simulink model "planta"  (R2025b)
settings: Solver=ode3  StartTime=0.0  StopTime=inf  FixedStep=0.001  RelTol=1e-3
values from neighbouring files (symbols this model uses):
  ah_max = 0.75    [init_plant_parameters.m]
  at_max = 0.80    (= 0.8)    [init_plant_parameters.m]
  bcx = 1.0e6    (= 1000000)    [init_plant_parameters.m]
  bcy = 10.0e6    (= 10000000)    [init_plant_parameters.m]
  bh_eq = bhm+bhd/ih^2    (= 18.0165289256)    [init_plant_parameters.m]
  bhb = 100e6    (= 100000000)    [init_plant_parameters.m]
  bhEb = 2.2e9    (= 2200000000)    [init_plant_parameters.m]
  bhwu = 150    [init_plant_parameters.m]
  bt = 90.0    (= 90)    [init_plant_parameters.m]
  bt_eq = btm+btd/it^2    (= 6.002)    [init_plant_parameters.m]
  btb = 5.0e6    (= 5000000)    [init_plant_parameters.m]
  btw = 3.0e3    (= 3000)    [init_plant_parameters.m]
  counter_limit = timeout/(Ts0*1000)    (= 1500)    [init_plant_parameters.m]
  envolvent = [ones(1,N_xt)]*38    [init_plant_parameters.m]
  g = 9.80665    [init_plant_parameters.m]
  Hc = 2.59    [init_plant_parameters.m]
  ih = 22.0    (= 22)    [init_plant_parameters.m]
  it = 30.0    (= 30)    [init_plant_parameters.m]
  Jh_eq = Jhm_hb+Jhd_hEb/ih^2    (= 37.8512396694)    [init_plant_parameters.m]
  Jt_eq = Jtm_tb+Jtd/it^2    (= 8.33333333333)    [init_plant_parameters.m]
  k_i_c = abs(polos_obs_c)^3    [init_plant_parameters.m]
  k_i_h = abs(polos_obs_h)^3    [init_plant_parameters.m]
  k_omega_c = 3 * abs(polos_obs_c)^2    [init_plant_parameters.m]
  k_omega_h = 3 * abs(polos_obs_h)^2-k_tita_h*bh_eq/Jh_eq    [init_plant_parameters.m]
  k_tita_c = 3 * abs(polos_obs_c)    [init_plant_parameters.m]
  k_tita_h = 3 * abs(polos_obs_h)-bh_eq/Jh_eq    [init_plant_parameters.m]
  Kcy = 1.8e9    (= 1800000000)    [init_plant_parameters.m]
  khwu = 236e6    (= 236000000)    [init_plant_parameters.m]
  Ki_c = (wn_t^2*Mt)/Kf    (= 320)    [init_plant_parameters.m]
  Ki_i = (wn_h^2)*Jh_eq    (= 2422.47933884)    [init_plant_parameters.m]
  Kp_c = (2*zitta_t*wn_t*Mt)/Kf    (= 1120)    [init_plant_parameters.m]
  Kp_i = 2*zitta_h*wn_h*Jh_eq    (= 1211.23966942)    [init_plant_parameters.m]
  Ktw = 480e3    (= 480000)    [init_plant_parameters.m]
  Lh0 = 110    [init_plant_parameters.m]
  lh_0 = Yt0-yh_0    (= 7)    [init_plant_parameters.m]
  Mc_max = 50000    [init_plant_parameters.m]
  Mc_min = 2000    [init_plant_parameters.m]
  Ms = 15000    [init_plant_parameters.m]
  Mt = 30000    [init_plant_parameters.m]
  P_nom = 956150    [init_plant_parameters.m]
  periodo_pulsos = 100    [init_plant_parameters.m]
  rhd = 0.75    [init_plant_parameters.m]
  rtd = 0.50    (= 0.5)    [init_plant_parameters.m]
  tau_hm = Ts2    (= 0.001)    [init_plant_parameters.m]
  tau_tm = Ts2    (= 0.001)    [init_plant_parameters.m]
  Thb_Max = 50e3    (= 50000)    [init_plant_parameters.m]
  ThEb_Max = 1.1e6    (= 1100000)    [init_plant_parameters.m]
  Thm_0 = 0    [init_plant_parameters.m]
  Thm_Max = 20e3    (= 20000)    [init_plant_parameters.m]
  titahm_0 = yl_0/(rhd/(2*ih))    (= 2228.19975108)    [init_plant_parameters.m]
  titatm_0 = xtd_0/(rtd/it)    (= 300)    [init_plant_parameters.m]
  Ts0 = 0.02    [init_plant_parameters.m]
  Ts1 = 0.02    [init_plant_parameters.m]
  Ttb_Max = 5.0e3    (= 5000)    [init_plant_parameters.m]
  Ttm_0 = 0    [init_plant_parameters.m]
  Ttm_Max = 4.0e3    (= 4000)    [init_plant_parameters.m]
  vh_0 = 0    [init_plant_parameters.m]
  vh_max = 3    [init_plant_parameters.m]
  vh_nom = 1.5    [init_plant_parameters.m]
  vt_0 = 0    [init_plant_parameters.m]
  vt_max = 4.0    (= 4)    [init_plant_parameters.m]
  Wc = 2.44    [init_plant_parameters.m]
  x_LIDAR = 3    [init_plant_parameters.m]
  xl_0 = 5    [init_plant_parameters.m]
  xt_0 = 5    [init_plant_parameters.m]
  xt_max = 50.0    (= 50)    [init_plant_parameters.m]
  xt_min = -30.0    (= -30)    [init_plant_parameters.m]
  xtd_0 = xt_0    (= 5)    [init_plant_parameters.m]
  yc0_vec_inicial = [ 0, 0, 1, 0, 0, 1, 0, 0, 0, 0, 0, 0, alt_borde,                   3, 5, 6, 3, 5, 6, 6, 4, 1, 1, -4, -5, -2, -1, 2, 6, 4, 2, 5,                   alt_borde] * Hc    [init_plant_parameters.m]
  yh_max = 40    [init_plant_parameters.m]
  yh_min = -20    [init_plant_parameters.m]
  yl_0 = Yt0 - l_0    (= 37.9806775752)    [init_plant_parameters.m]
  Yt0 = 45.0    (= 45)    [init_plant_parameters.m]
  zitta = 0.5    [init_plant_parameters.m]
undefined symbols (not defined in the file or in its folder): DiscIntNeverNeededParam
libraries: sl3dlib x1, dspnetwork x1
(part 1 of 2)
settings Model: SimulationMode=accelerator  PacingRate=2  Creator=lauta  LastModifiedBy=bruno

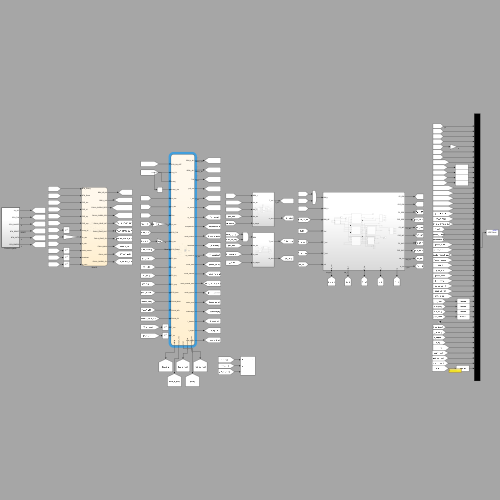
[thumbnail: Simulink's stored preview of the top-level diagram]
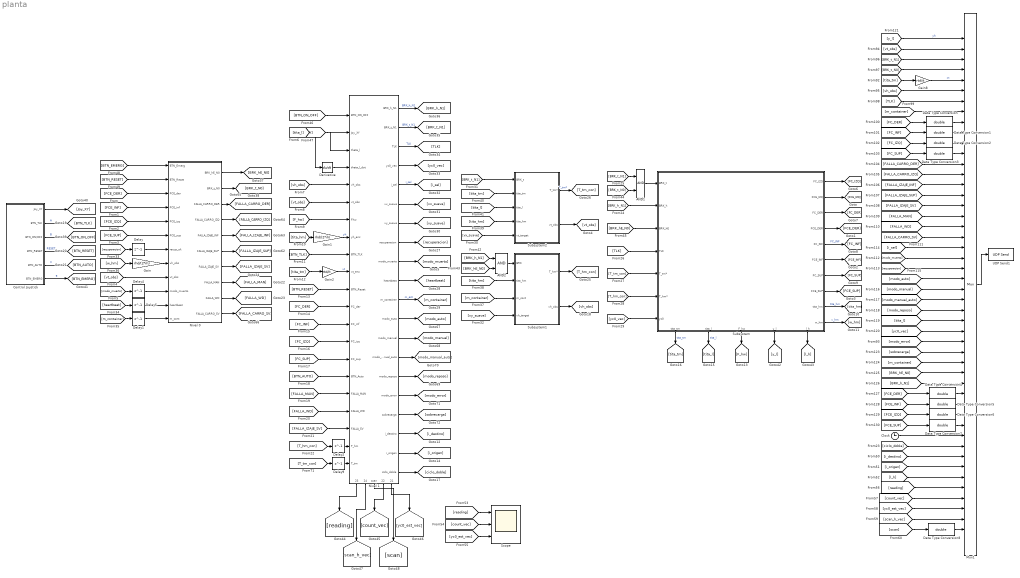
== system planta ==
  AND1 : Logic  IconShape=distinctive  AllPortsSameDT=off  OutDataTypeStr=boolean
  AND2 : Logic  IconShape=distinctive  AllPortsSameDT=off  OutDataTypeStr=boolean
  Clock : Clock
  "Control Joystick " : Subsystem  TreatAsAtomicUnit=on  SystemSampleTime=tau_hm
  Data Type Conversion{,1..8} (9 alike) : DataTypeConversion  OutDataTypeStr=double  SaturateOnIntegerOverflow=off  RndMeth=Floor
  Delay{,1..2,4..5,9} (6 alike) : Delay  DelayLength=1  InputProcessing=Columns as channels (frame based)  SampleTime=Ts0
  Derivative : Derivative
  Gain : Gain  Gain=rhd/(2*ih)
  Gain1 : Gain  Gain=rhd/(2*ih)
  Gain2 : Gain  Gain=rtd/it
  Gain8 : Gain  Gain=rtd/it
  Mux1 : Mux  Inputs=48
  Nivel 0 : Stateflow chart  TreatAsAtomicUnit=on  SystemSampleTime=Ts0
  Nivel 1 : Stateflow chart  TreatAsAtomicUnit=on  SystemSampleTime=Ts1
      settings: PortSchema="{\"entries\":[{\"content\":{\"sides\":[{\"content\":{\"connectorIds\":[\"In1\",\"In2\",\"In3\",\"In4\",\"In5\",\"In6\",\"In7\",\"In8\",\"In9\",\"In10\",\"In11\",\"In12\",\"In13\",\"In14\",\"In15\",\"In16\",\"In17\",\"In18\",\"In19\",\"In20\",\"In21\"]},\"type\":\"ConnectorPlacement.EquallySpacedRectSide\",\"uuid\":\"f9309f7f-3c54-46e4-8c5b-2437500e737a\"},{\"content\":{\"connectorIds\":[\"Out1\",\"Out2\",\"Out3\",\"Out4\",\"Out5\",\"Out6\",\"Out7\",\"Out8\",\"Out9\",\"Out10\",\"Out11\",\"Out12\",\"Out13\",\"Out14\",\"Out15\",\"Out16\",\"Out17\",\"Out18\",\"Out19\",\"Out20\"],\"side\":\"RIGHT\"},\"type\":\"ConnectorPlacement.EquallySpacedRectSide\",\"uuid\":\"ccb321bc-00c9-4449-9a3e-5435c9b39512\"},{\"content\":{\"side\":\"TOP\"},\"type\":\"ConnectorPlacement.EquallySpacedRectSide\",\"uuid\":\"3099bf00-db3f-4e40-be81-3cc0981b79ca\"},{\"content\":{\"connectorIds\":[\"Out23\",\"Out24\",\"Out25\",\"Out22\",\"Out21\"],\"side\":\"BOTTOM\"},\"type\":\"ConnectorPlacement.EquallySpacedRectSide\",\"uuid\":\"36423b9f-354b-4379-ba2c-4a5a21c34b61\"}]},\"type\":\"ConnectorPlacement.EquallySpacedConnector\",\"uuid\":\"738d8a71-e82f-4c2f-ab09-6d96e2c2ffc9\"}],\"packageUris\":[\"http://schema.mathworks.com/mf0/Connector/R2020b\"],\"version\":\"1.0\"}"
  Scope : Scope  NumInputPorts=3
      settings: ActiveDisplayYMinimum=-212.88770278621519  ActiveDisplayYMaximum=339.27135541787879
  Subsystem : Subsystem
      settings: PortSchema="{\"entries\":[{\"content\":{\"sides\":[{\"content\":{\"connectorIds\":[\"In1\",\"In2\",\"In3\",\"In4\",\"In5\",\"In6\",\"In7\"]},\"type\":\"ConnectorPlacement.EquallySpacedRectSide\",\"uuid\":\"af149f61-d672-449c-a7fb-5624cb810af3\"},{\"content\":{\"connectorIds\":[\"Out1\",\"Out2\",\"Out3\",\"Out4\",\"Out5\",\"Out6\",\"Out7\",\"Out8\",\"Out9\",\"Out10\"],\"side\":\"RIGHT\"},\"type\":\"ConnectorPlacement.EquallySpacedRectSide\",\"uuid\":\"108c8060-9c99-461a-9367-2154718b4d28\"},{\"content\":{\"side\":\"TOP\"},\"type\":\"ConnectorPlacement.EquallySpacedRectSide\",\"uuid\":\"cb8fd5b9-c875-48a1-bd6c-0e8918880b0e\"},{\"content\":{\"connectorIds\":[\"Out11\",\"Out12\",\"Out13\",\"Out14\",\"Out15\"],\"side\":\"BOTTOM\"},\"type\":\"ConnectorPlacement.EquallySpacedRectSide\",\"uuid\":\"417db1a2-cc41-4820-881b-53f0e9bd83f8\"}]},\"type\":\"ConnectorPlacement.EquallySpacedConnector\",\"uuid\":\"d40848f9-2d56-455f-ab83-092311f7e026\"}],\"packageUris\":[\"http://schema.mathworks.com/mf0/Connector/R2020b\"],\"version\":\"1.0\"}"
  Subsystem1 : Subsystem
  Subsystem2 : Subsystem
  UDP Send1 : dspnetwork/UDP Send  remoteURL='127.0.0.1'  remotePort=1234  localURL='0.0.0.0'  localPortSource=Automatically determine  localPort=-1  sendBufferSize=8192  sampletime=-1  blockPlatform=HOST  separateLengthPort=0
  wires:
  Subsystem2/1(T_tm*) -> [T_tm_con]  "T_tm*"
  Subsystem/12(tita_l) -> [tita_l]  "tita_l"
  Subsystem1/1(T_hm*) -> [T_hm_con]
  Subsystem/11(tita_tm) -> [tita_tm]  "tita_tm"
  Subsystem/9(tita_hm) -> [tita_hm]  "tita_hm"
  Nivel 1/1(BRK_h_N1) -> [BRK_h_N1]  "BRK_h_N1"
  Nivel 1/2(BRK_t_N1) -> [BRK_t_N1]  "BRK_t_N1"
  "Control Joystick "/1(Joy_XY) -> [Joy_XY]
  Subsystem2/2(vt_obs) -> [vt_obs]
  Subsystem1/2(vh_obs) -> [vh_obs]
  Derivative/1 -> Nivel 1/4(theta_l_dot)
  Subsystem/13(F_hw) -> [F_hw]
  Nivel 1/3(TLK) -> [TLK]  "TLK"
  "Control Joystick "/2(BTN_TLK) -> [BTN_TLK]  "A"
  Nivel 1/4(yc0_vec) -> [yc0_vec]
  Nivel 1/11(m_container) -> [m_container]  "m_est"
  "Control Joystick "/4(BTN_RESET) -> [BTN_RESET]  "RESET"
  Subsystem/3(FC_DER) -> [FC_DER]
  Subsystem/5(FC_INF) -> [FC_INF]  "FC_INF"
  Subsystem/7(FC_SUP) -> [FC_SUP]
  "Control Joystick "/5(BTN_AUTO) -> [BTN_AUTO]  "X"
  Nivel 1/6(vx_suave) -> [vx_suave]
  Nivel 1/7(vy_suave) -> [vy_suave]
  "Control Joystick "/6(BTN_EMERG) -> [BTN_EMERG]  "9"
  Nivel 1/8(recuperacion) -> [recuperacion]
  Subsystem/10(w_hm) -> [w_hm]  "v_hm"
  Gain/1 -> Nivel 0/8(vh_obs)
  AND1/1 -> Subsystem/1(BRK_t)
  Nivel 0/2(BRK_t_N0) -> [BRK_t_N0]
  Subsystem/2(FCE_IZQ) -> [FCE_IZQ]
  Subsystem/4(FCE_DER) -> [FCE_DER]
  Subsystem/6(FCE_INF) -> [FCE_INF]
  Subsystem/8(FCE_SUP) -> [FCE_SUP]
  [FCE_DER] -> Nivel 0/3(FCE_der)
  [FCE_INF] -> Nivel 0/4(FCE_inf)
  [FCE_IZQ] -> Nivel 0/5(FCE_izq)
  [FCE_SUP] -> Nivel 0/6(FCE_sup)
  Nivel 0/8(FALLA_MAN) -> [FALLA_MAN]
  Nivel 0/9(FALLA_WD) -> [FALLA_WD]
  Nivel 0/7(FALLA_IZAJE_SV) -> [FALLA_IZAJE_SV]
  Delay/1 -> Nivel 0/7(recup_ok)
  Delay1/1 -> Nivel 0/12(m_cont)
  [vt_obs] -> Nivel 0/9(vt_obs)
  "Control Joystick "/3(BTN_ON/OFF) -> [BTN_ON_OFF]  "B"
  Delay2/1 -> Nivel 1/20(T_hm)
  Delay9/1 -> Nivel 1/21(T_tm)
  Nivel 1/9(modo_muerto) -> [modo_muerto]
  [modo_muerto] -> Delay4/1
  Nivel 1/10(heartbeat) -> [heartbeat]
  Delay4/1 -> Nivel 0/10(modo_muerto)
  Delay5/1 -> Nivel 0/11(heartbeat)
  [tita_l] -> Derivative/1, Nivel 1/3(theta_l)
  [vh_obs] -> Nivel 1/5(vh_obs)
  [vt_obs] -> Nivel 1/6(vt_obs)
  [F_hw] -> Nivel 1/7(Fhw)
  [tita_hm] -> Gain1/1
  Gain1/1 -> Nivel 1/8(yh_enc)  "yh"
  [BTN_TLK] -> Nivel 1/9(BTN_TLK)
  [tita_tm] -> Gain2/1
  Gain2/1 -> Nivel 1/10(xt_enc)  "xt"
  [BTN_RESET] -> Nivel 1/11(BTN_Reset)
  [FC_DER] -> Nivel 1/12(FC_der)
  [FC_INF] -> Nivel 1/13(FC_inf)
  [FC_IZQ] -> Nivel 1/14(FC_izq)
  [FC_SUP] -> Nivel 1/15(FC_sup)
  [BTN_AUTO] -> Nivel 1/16(BTN_Auto)
  [FALLA_MAN] -> Nivel 1/17(FALLA_MAN)
  [FALLA_WD] -> Nivel 1/18(FALLA_WD)
  [FALLA_IZAJE_SV] -> Nivel 1/19(FALLA_SV)
  [T_hm_con] -> Delay2/1
  [T_tm_con] -> Delay9/1
  Nivel 1/5(i_sel) -> [i_sel]  "i_sel"
  [BRK_h_N1] -> Subsystem/2(BRK_h)
  [BRK_t_N1] -> AND1/1
  [TLK] -> Subsystem/4(TLK)
  [T_tm_con] -> Subsystem/5(T_tm*)
  [T_hm_con] -> Subsystem/6(T_hm*)
  [yc0_vec] -> Subsystem/7(yc0)
  [vx_suave] -> Subsystem2/5(vt_target)
  [BRK_t_N1] -> Subsystem2/1(BRK_t)
  [vy_suave] -> Subsystem1/4(vh_target)
  [recuperacion] -> Delay/1
  [heartbeat] -> Delay5/1
  [m_container] -> Delay1/1
  [w_hm] -> Gain/1
  [m_container] -> Subsystem1/3(m_cont)
  [tita_hm] -> Subsystem1/2(tita_hm)
  [tita_hm] -> Subsystem2/4(tita_hm)
  [tita_tm] -> Subsystem2/2(tita_tm)
  [tita_l] -> Subsystem2/3(tita_l)
  [BRK_h_N1] -> AND2/1
  AND2/1 -> Subsystem1/1(BRK)
  Nivel 0/1(BRK_hE_N0) -> [BRK_hE_N0]
  [BRK_hE_N0] -> AND2/2
  [BRK_t_N0] -> AND1/2
  [BRK_hE_N0] -> Subsystem/3(BRK_hE)
  [BTN_ON_OFF] -> Nivel 1/1(BTN_ON_OFF)
  [Joy_XY] -> Nivel 1/2(Joy_XY)
  [BTN_EMERG] -> Nivel 0/1(BTN_Emerg)
  [BTN_RESET] -> Nivel 0/2(BTN_Reset)
  Subsystem/14(y_l) -> [y_l]
  Nivel 0/3(FALLA_CARRO_DER) -> [FALLA_CARRO_DER]
  Nivel 0/4(FALLA_CARRO_IZQ) -> [FALLA_CARRO_IZQ]
  Nivel 0/5(FALLA_IZAJE_INF) -> [FALLA_IZAJE_INF]
  Nivel 0/6(FALLA_IZAJE_SUP) -> [FALLA_IZAJE_SUP]
  Nivel 0/10(FALLA_CARRO_SV) -> [FALLA_CARRO_SV]
  Mux1/1 -> UDP Send1/1
  Nivel 1/12(modo_auto) -> [modo_auto]
  Nivel 1/13(modo_manual) -> [modo_manual]
  Nivel 1/14(modo_manual_auto) -> [modo_manual_auto]
  Nivel 1/15(modo_reposo) -> [modo_reposo]
  [y_l] -> Mux1/1  "yh"
  [vt_obs] -> Mux1/2
  [BRK_t_N1] -> Mux1/3
  [BRK_t_N0] -> Mux1/4
  [vh_obs] -> Mux1/6
  [TLK] -> Mux1/7
  [m_container] -> Mux1/8
  [FC_INF] -> Data Type Conversion1/1
  [FC_SUP] -> Data Type Conversion3/1
  [FALLA_CARRO_DER] -> Mux1/13
  [FALLA_CARRO_IZQ] -> Mux1/14
  [FALLA_IZAJE_INF] -> Mux1/15
  [FALLA_IZAJE_SUP] -> Mux1/16
  [FALLA_IZAJE_SV] -> Mux1/17
  [FALLA_MAN] -> Mux1/18
  [FALLA_WD] -> Mux1/19
  [FALLA_CARRO_SV] -> Mux1/20
  [i_sel] -> Mux1/21
  [modo_muerto] -> Mux1/22
  [recuperacion] -> Mux1/23
  [modo_auto] -> Mux1/24
  [modo_manual] -> Mux1/25
  [modo_manual_auto] -> Mux1/26
  [modo_reposo] -> Mux1/27
  [tita_tm] -> Gain8/1
  Gain8/1 -> Mux1/5  "xt"
  [FC_IZQ] -> Data Type Conversion2/1
  [FC_DER] -> Data Type Conversion/1
  Data Type Conversion/1 -> Mux1/9
  Subsystem/1(FC_IZQ) -> [FC_IZQ]
  Data Type Conversion1/1 -> Mux1/10
  Data Type Conversion2/1 -> Mux1/11
  Data Type Conversion3/1 -> Mux1/12
  [tita_l] -> Mux1/28
  [yc0_vec] -> Mux1/29
  Nivel 1/16(modo_error) -> [modo_error]
  [modo_error] -> Mux1/30
  Nivel 1/17(sobrecarga) -> [sobrecarga]
  [sobrecarga] -> Mux1/31
  [m_container] -> Mux1/32
  [BRK_hE_N0] -> Mux1/33
  [BRK_h_N1] -> Mux1/34
  [FCE_DER] -> Data Type Conversion4/1
  [FCE_INF] -> Data Type Conversion5/1
  [FCE_IZQ] -> Data Type Conversion6/1
  [FCE_SUP] -> Data Type Conversion7/1
  Data Type Conversion5/1 -> Mux1/36
  Data Type Conversion6/1 -> Mux1/37
  Data Type Conversion7/1 -> Mux1/38
  Data Type Conversion4/1 -> Mux1/35
  Clock/1 -> Mux1/39
  Nivel 1/18(i_destino) -> [i_destino]
  Nivel 1/19(i_origen) -> [i_origen]
  Nivel 1/20(ciclo_doble) -> [ciclo_doble]
  [ciclo_doble] -> Mux1/40
  [i_destino] -> Mux1/41
  [i_origen] -> Mux1/42
  Subsystem/15(l_h) -> [l_h]
  [l_h] -> Mux1/43
  [reading] -> Scope/1
  [count_vec] -> Scope/2
  [yc0_est_vec] -> Scope/3
  [reading] -> Mux1/44
  [count_vec] -> Mux1/45
  [yc0_est_vec] -> Mux1/46
  Nivel 1/23(reading) -> [reading]
  Nivel 1/22(count_vec) -> [count_vec]
  Nivel 1/21(yc0_est_vec) -> [yc0_est_vec]
  Nivel 1/24(scan_h_vec) -> [scan_h_vec]
  [scan_h_vec] -> Mux1/47
  Nivel 1/25(scan) -> [scan]
  [scan] -> Data Type Conversion8/1
  Data Type Conversion8/1 -> Mux1/48

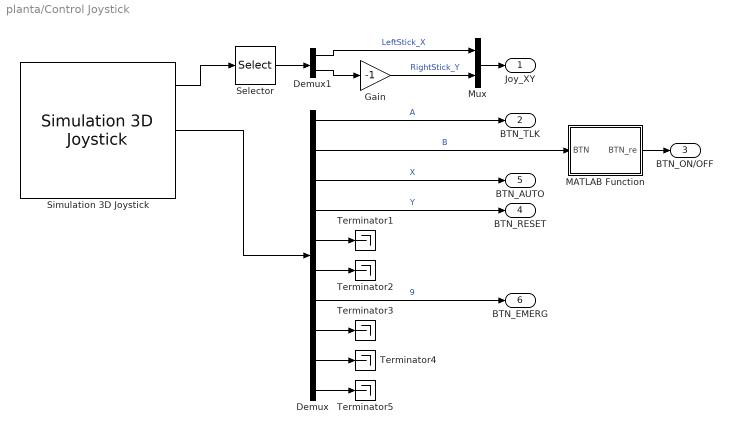
== system planta/Control Joystick  ==
  Demux : Demux  Outputs=10
  Demux1 : Demux  Outputs=2
  Gain : Gain  Gain=-1
  MATLAB Function : MATLAB Function  TreatAsAtomicUnit=on
  Mux : Mux  Inputs=2
  Selector : Selector  InputPortWidth=5  IndexOptions=Index vector (dialog)  Indices=[1 5]  OutputSizes=1
  Simulation 3D Joystick : sl3dlib/Simulation 3D/Hardware Interface/Simulation 3D Joystick  joyid=1  adjustports=on  forcefeed=off
  Terminator{1..5} (5 alike) : Terminator
  Joy_XY : Outport
  BTN_TLK : Outport  Port=2
  BTN_ON/OFF : Outport  Port=3
  BTN_RESET : Outport  Port=4
  BTN_AUTO : Outport  Port=5
  BTN_EMERG : Outport  Port=6
  wires:
  Demux/1 -> BTN_TLK/1  "A"
  Demux1/2 -> Gain/1
  Demux1/1 -> Mux/1  "LeftStick_X"
  Selector/1 -> Demux1/1
  Simulation 3D Joystick/1 -> Selector/1
  Gain/1 -> Mux/2  "RightStick_Y"
  Simulation 3D Joystick/2 -> Demux/1
  Demux/2 -> MATLAB Function/1(BTN)  "B"
  Demux/3 -> BTN_AUTO/1  "X"
  Demux/4 -> BTN_RESET/1  "Y"
  Mux/1 -> Joy_XY/1
  Demux/5 -> Terminator1/1
  Demux/6 -> Terminator2/1
  Demux/8 -> Terminator3/1
  Demux/9 -> Terminator4/1
  Demux/10 -> Terminator5/1
  Demux/7 -> BTN_EMERG/1  "9"
  MATLAB Function/1(BTN_re) -> BTN_ON/OFF/1

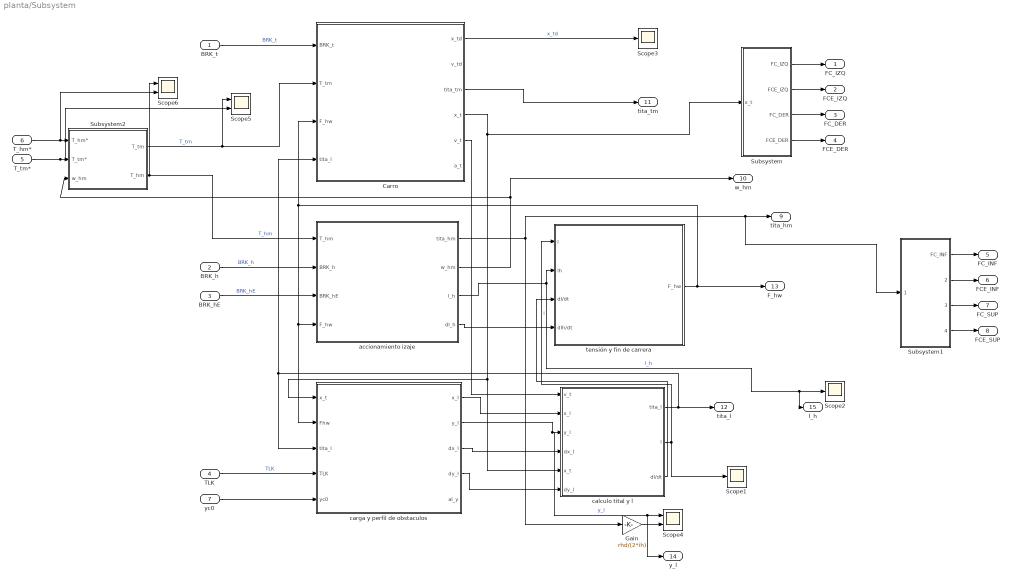
== system planta/Subsystem ==
  BRK_t : Inport
  BRK_h : Inport  Port=2
  BRK_hE : Inport  Port=3
  TLK : Inport  Port=4
  T_tm* : Inport  Port=5
  T_hm* : Inport  Port=6
  yc0 : Inport  Port=7
  Carro : Subsystem
  Gain : Gain  Gain=rhd/(2*ih)
  Scope1 : Scope
      settings: ActiveDisplayYMinimum=-3.1438  ActiveDisplayYMaximum=28.29416  DataLoggingVariableName=ScopeData5
  Scope2 : Scope
      settings: ActiveDisplayYMinimum=19.873309767116591  ActiveDisplayYMaximum=50.479762765379171  DataLoggingVariableName=ScopeData6
  Scope3 : Scope
      settings: ActiveDisplayYMinimum=-36.0687664182162  ActiveDisplayYMaximum=31.78541849091291
  Scope4 : Scope  NumInputPorts=2
      settings: ActiveDisplayYMinimum=31.554051944720545  ActiveDisplayYMaximum=41.717948866314323  DataLoggingVariableName=ScopeData13
  Scope5 : Scope  NumInputPorts=2
      settings: ActiveDisplayYMinimum=2216.0147211124222  ActiveDisplayYMaximum=3994.0783191721102  DataLoggingVariableName=ScopeData12
  Scope6 : Scope  NumInputPorts=2
      settings: ActiveDisplayYMinimum=-18675.827607289168  ActiveDisplayYMaximum=162181.63787626589  DataLoggingVariableName=ScopeData17
  Subsystem : Subsystem
  Subsystem1 : Subsystem
  Subsystem2 : Subsystem
  accionamiento izaje : Subsystem
  calculo tital y l : Subsystem
  carga y perfil de obstaculos : Subsystem
  tensión y fin de carrera : Subsystem
  FC_IZQ : Outport
  FCE_IZQ : Outport  Port=2
  FC_DER : Outport  Port=3
  FCE_DER : Outport  Port=4
  FC_INF : Outport  Port=5
  FCE_INF : Outport  Port=6
  FC_SUP : Outport  Port=7
  FCE_SUP : Outport  Port=8
  tita_hm : Outport  Port=9
  w_hm : Outport  Port=10
  tita_tm : Outport  Port=11
  tita_l : Outport  Port=12
  F_hw : Outport  Port=13
  y_l : Outport  Port=14
  l_h : Outport  Port=15
  wires:
  Subsystem2/2(T_hm) -> Scope6/1, accionamiento izaje/1(T_hm)  "T_hm"
  Carro/1(x_td) -> Scope3/1  "x_td"
  Carro/5(v_t) -> calculo tital y l/1(v_t)
  calculo tital y l/3(dl/dt) -> tensión y fin de carrera/3(dl/dt)
  carga y perfil de obstaculos/3(dx_l) -> calculo tital y l/4(dx_l)
  tensión y fin de carrera/1(F_hw) -> carga y perfil de obstaculos/2(Fhw), accionamiento izaje/4(F_hw), Carro/3(F_hw), F_hw/1
  carga y perfil de obstaculos/1(x_l) -> calculo tital y l/2(x_l)
  BRK_t/1 -> Carro/1(BRK_t)  "BRK_t"
  Subsystem2/1(T_tm) -> Scope5/1, Carro/2(T_tm)  "T_tm"
  BRK_hE/1 -> accionamiento izaje/3(BRK_hE)  "BRK_hE"
  BRK_h/1 -> accionamiento izaje/2(BRK_h)  "BRK_h"
  accionamiento izaje/3(l_h) -> l_h/1, Scope2/1, tensión y fin de carrera/2(lh)  "l_h"
  calculo tital y l/1(tita_l) -> tita_l/1, carga y perfil de obstaculos/3(tita_l), Carro/4(tita_l)
  carga y perfil de obstaculos/4(dy_l) -> calculo tital y l/6(dy_l)
  Carro/4(x_t) -> carga y perfil de obstaculos/1(x_t), calculo tital y l/5(x_t), Subsystem/1(x_t)
  carga y perfil de obstaculos/2(y_l) -> y_l/1, Scope4/1, calculo tital y l/3(y_l)  "y_l"
  calculo tital y l/2(l) -> Scope1/1, tensión y fin de carrera/1(l)  "l"
  accionamiento izaje/1(tita_hm) -> Gain/1, Subsystem1/1(tita_hm), tita_hm/1
  TLK/1 -> carga y perfil de obstaculos/4(TLK)  "TLK"
  Carro/3(tita_tm) -> tita_tm/1
  accionamiento izaje/2(w_hm) -> Subsystem2/3(w_hm), w_hm/1
  T_hm*/1 -> Scope6/2, Subsystem2/1(T_hm*)
  T_tm*/1 -> Scope5/2, Subsystem2/2(T_tm*)
  accionamiento izaje/4(dl_h) -> tensión y fin de carrera/4(dlh/dt)
  yc0/1 -> carga y perfil de obstaculos/5(yc0)
  Subsystem/1(FC_IZQ) -> FC_IZQ/1
  Subsystem/2(FCE_IZQ) -> FCE_IZQ/1
  Subsystem/3(FC_DER) -> FC_DER/1
  Subsystem/4(FCE_DER) -> FCE_DER/1
  Subsystem1/1(FC_INF) -> FC_INF/1
  Subsystem1/2(FCE_INF) -> FCE_INF/1
  Subsystem1/3(FC_SUP) -> FC_SUP/1
  Subsystem1/4(FCE_SUP) -> FCE_SUP/1
  Gain/1 -> Scope4/2

== system planta/Subsystem1 ==
  BRK : Inport
  tita_hm : Inport  Port=2
  m_cont : Inport  Port=3
  vh_target : Inport  Port=4
  Controlador de Velocidad : Subsystem  TreatAsAtomicUnit=on  SystemSampleTime=tau_hm
  Delay2 : Delay  DelayLength=1  InitialCondition=Thm_0
  Modulación de la Referencia : Subsystem  TreatAsAtomicUnit=on  SystemSampleTime=tau_tm
  Observador de estado : Subsystem  TreatAsAtomicUnit=on  SystemSampleTime=tau_hm
  Scope : Scope
      settings: ActiveDisplayYMinimum=-0.34044660881355743  ActiveDisplayYMaximum=0.29766878557385207  DataLoggingVariableName=ScopeData22
  Scope1 : Scope
      settings: ActiveDisplayYMinimum=2409.3798864876212  ActiveDisplayYMaximum=2546.7876456481149  DataLoggingVariableName=ScopeData23
  Scope2 : Scope
      settings: ActiveDisplayYMinimum=-0.0013706448423018264  ActiveDisplayYMaximum=0.0033174735734584049  DataLoggingVariableName=ScopeData24
  T_hm* : Outport
  vh_obs : Outport  Port=2
  wires:
  Delay2/1 -> Observador de estado/2(Thm_ref)
  Modulación de la Referencia/1(vh_ref) -> Scope/1, Controlador de Velocidad/3(vh_ref)
  m_cont/1 -> Controlador de Velocidad/1(m_container)
  BRK/1 -> Controlador de Velocidad/2(BRK)
  Controlador de Velocidad/1(T_hm*) -> Scope1/1, T_hm*/1, Delay2/1
  Observador de estado/1(vh_obs) -> Scope2/1, vh_obs/1, Controlador de Velocidad/4(vh_obs)
  tita_hm/1 -> Observador de estado/1(yh_enc)
  vh_target/1 -> Modulación de la Referencia/1(vh)

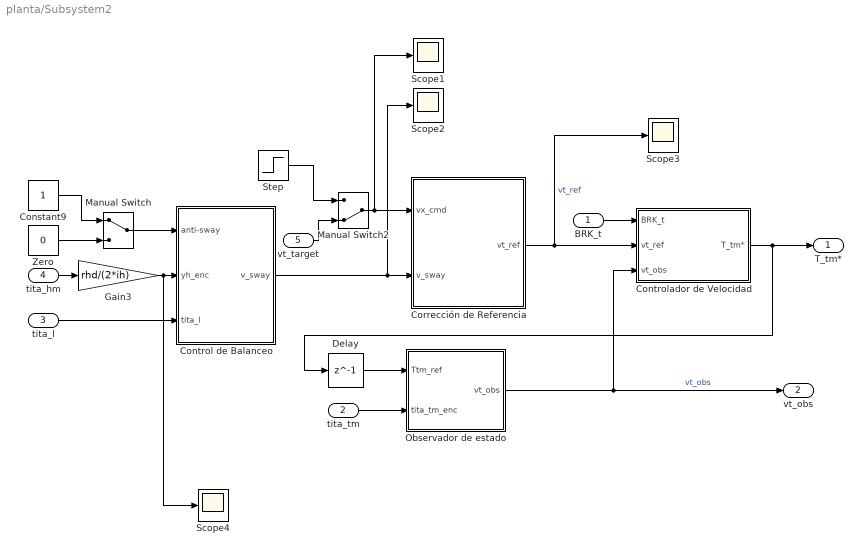
== system planta/Subsystem2 ==
  BRK_t : Inport
  tita_tm : Inport  Port=2
  tita_l : Inport  Port=3
  tita_hm : Inport  Port=4
  vt_target : Inport  Port=5
  Constant9 : Constant
  Control de Balanceo : Subsystem
  Controlador de Velocidad : Subsystem
  Corrección de Referencia : Subsystem
  Delay : Delay  DelayLength=1  InitialCondition=Ttm_0
  Gain3 : Gain  Gain=rhd/(2*ih)
  Manual Switch : ManualSwitch
  Manual Switch2 : ManualSwitch  CurrentSetting=0
  Observador de estado : Subsystem  TreatAsAtomicUnit=on  SystemSampleTime=tau_hm
  Scope{1..4} (4 alike) : Scope
      Scope1 settings: ActiveDisplayYMinimum=-0.5858905301065096  ActiveDisplayYMaximum=1.1762100589007232  DataLoggingVariableName=ScopeData14
      Scope2 settings: ActiveDisplayYMinimum=-0.71026747882004693  ActiveDisplayYMaximum=0.0886681616928574  DataLoggingVariableName=ScopeData15
      Scope3 settings: ActiveDisplayYMinimum=-0.6534407131284351  ActiveDisplayYMaximum=0.071217464207534387  DataLoggingVariableName=ScopeData16
      Scope4 settings: ActiveDisplayYMinimum=-69.230490323598147  ActiveDisplayYMaximum=39.5853363197014  DataLoggingVariableName=ScopeData20
  Step : Step  Time=2  SampleTime=0
  Zero : Constant  Value=0  OutDataTypeStr=Inherit: Inherit via back propagation
  T_tm* : Outport
  vt_obs : Outport  Port=2
  wires:
  Corrección de Referencia/1(vt_ref) -> Scope3/1, Controlador de Velocidad/2(vt_ref)  "vt_ref"
  Controlador de Velocidad/1(T_tm*) -> T_tm*/1, Delay/1
  Observador de estado/1(vt_obs) -> Controlador de Velocidad/3(vt_obs), vt_obs/1  "vt_obs"
  Control de Balanceo/1(v_sway) -> Scope2/1, Corrección de Referencia/2(v_sway)
  tita_tm/1 -> Observador de estado/2(tita_tm_enc)
  tita_l/1 -> Control de Balanceo/3(tita_l)
  Delay/1 -> Observador de estado/1(Ttm_ref)
  BRK_t/1 -> Controlador de Velocidad/1(BRK_t)
  tita_hm/1 -> Gain3/1
  Manual Switch/1 -> Control de Balanceo/1(anti-sway)
  Zero/1 -> Manual Switch/2
  Constant9/1 -> Manual Switch/1
  Gain3/1 -> Scope4/1, Control de Balanceo/2(yh_enc)
  Manual Switch2/1 -> Scope1/1, Corrección de Referencia/1(vx_cmd)
  vt_target/1 -> Manual Switch2/2
  Step/1 -> Manual Switch2/1

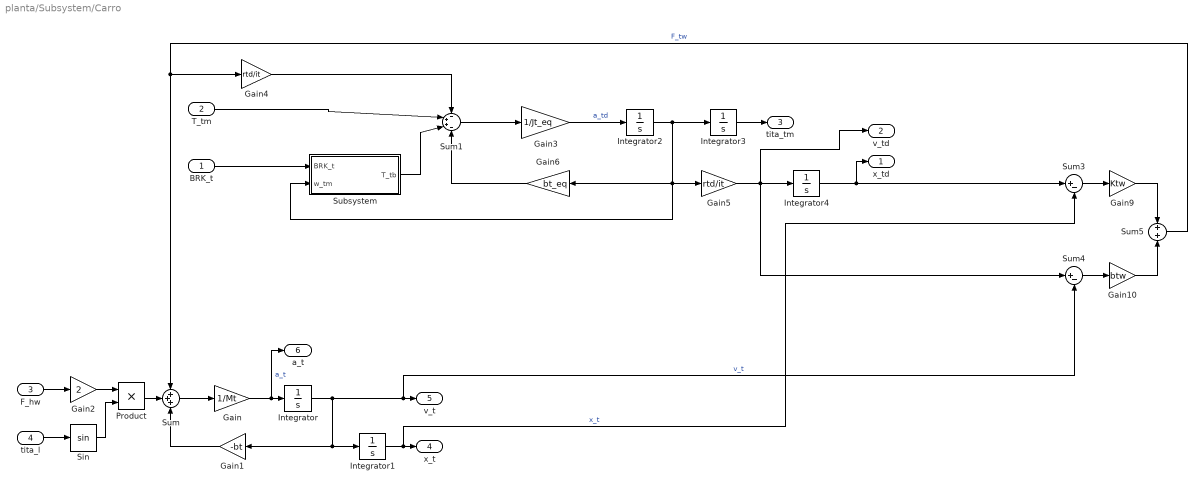
== system planta/Subsystem/Carro ==
  BRK_t : Inport
  T_tm : Inport  Port=2
  F_hw : Inport  Port=3
  tita_l : Inport  Port=4
  Gain : Gain  Gain=1/Mt
  Gain1 : Gain  Gain=-bt
  Gain10 : Gain  Gain=btw
  Gain2 : Gain  Gain=2
  Gain3 : Gain  Gain=1/Jt_eq
  Gain4 : Gain  Gain=rtd/it
  Gain5 : Gain  Gain=rtd/it
  Gain6 : Gain  Gain=bt_eq
  Gain9 : Gain  Gain=Ktw
  Integrator : Integrator
  Integrator1 : Integrator  InitialCondition=xt_0
  Integrator2 : Integrator
  Integrator3 : Integrator  InitialCondition=titatm_0
  Integrator4 : Integrator  InitialCondition=xtd_0
  Product : Product
  Sin : Trigonometry
  Subsystem : Subsystem
  Sum : Sum  Inputs=+++
  Sum1 : Sum  Inputs=-++-
  Sum3 : Sum  Inputs=|+-
  Sum4 : Sum  Inputs=|+-
  Sum5 : Sum
  x_td : Outport
  v_td : Outport  Port=2
  tita_tm : Outport  Port=3
  x_t : Outport  Port=4
  v_t : Outport  Port=5
  a_t : Outport  Port=6
  wires:
  F_hw/1 -> Gain2/1
  tita_l/1 -> Sin/1
  Sin/1 -> Product/2
  Product/1 -> Sum/2
  Integrator/1 -> Integrator1/1, Gain1/1, Sum4/2, v_t/1  "v_t"
  Gain2/1 -> Product/1
  Sum5/1 -> Sum/1, Gain4/1  "F_tw"
  Sum/1 -> Gain/1
  Gain1/1 -> Sum/3
  Gain/1 -> a_t/1, Integrator/1  "a_t"
  Integrator1/1 -> Sum3/2, x_t/1  "x_t"
  Sum1/1 -> Gain3/1
  Gain3/1 -> Integrator2/1  "a_td"
  Gain4/1 -> Sum1/1
  T_tm/1 -> Sum1/2
  BRK_t/1 -> Subsystem/1(BRK_t)
  Gain9/1 -> Sum5/1
  Integrator3/1 -> tita_tm/1
  Integrator2/1 -> Gain6/1, Subsystem/2(w_tm), Gain5/1, Integrator3/1
  Sum3/1 -> Gain9/1
  Gain10/1 -> Sum5/2
  Sum4/1 -> Gain10/1
  Subsystem/1(T_tb) -> Sum1/3
  Gain6/1 -> Sum1/4
  Gain5/1 -> v_td/1, Sum4/1, Integrator4/1
  Integrator4/1 -> x_td/1, Sum3/1

== system planta/Subsystem/Subsystem ==
  x_t : Inport
  Constant1 : Constant  Value=xt_min
  Constant2 : Constant  Value=xt_min-0.5
  Constant3 : Constant  Value=xt_max
  Constant4 : Constant  Value=xt_max+0.5
  Relational Operator : RelationalOperator  Operator=<=  OutDataTypeStr=boolean  RndMeth=Simplest  InputSameDT=off
  Relational Operator1 : RelationalOperator  Operator=<=  OutDataTypeStr=boolean  RndMeth=Simplest  InputSameDT=off
  Relational Operator2 : RelationalOperator  OutDataTypeStr=boolean  RndMeth=Simplest  InputSameDT=off
  Relational Operator3 : RelationalOperator  OutDataTypeStr=boolean  RndMeth=Simplest  InputSameDT=off
  FC_IZQ : Outport
  FCE_IZQ : Outport  Port=2
  FC_DER : Outport  Port=3
  FCE_DER : Outport  Port=4
  wires:
  Constant3/1 -> Relational Operator2/2
  Relational Operator3/1 -> FCE_DER/1
  x_t/1 -> Relational Operator3/1, Relational Operator2/1, Relational Operator/1, Relational Operator1/1  "x_t"
  Relational Operator/1 -> FC_IZQ/1
  Constant2/1 -> Relational Operator1/2
  Relational Operator1/1 -> FCE_IZQ/1
  Constant1/1 -> Relational Operator/2
  Relational Operator2/1 -> FC_DER/1
  Constant4/1 -> Relational Operator3/2

== system planta/Subsystem/Subsystem1 ==
  tita_hm : Inport
  Constant10 : Constant  Value=yh_max+0.5
  Constant7 : Constant  Value=yh_min
  Constant8 : Constant  Value=yh_min-0.5
  Constant9 : Constant  Value=yh_max
  Gain3 : Gain  Gain=rhd/(2*ih)
  Relational Operator1 : RelationalOperator  Operator=<=  OutDataTypeStr=boolean  RndMeth=Simplest  InputSameDT=off
  Relational Operator2 : RelationalOperator  Operator=<=  OutDataTypeStr=boolean  RndMeth=Simplest  InputSameDT=off
  Relational Operator3 : RelationalOperator  OutDataTypeStr=boolean  RndMeth=Simplest  InputSameDT=off
  Relational Operator4 : RelationalOperator  OutDataTypeStr=boolean  RndMeth=Simplest  InputSameDT=off
  FC_INF : Outport
  FCE_INF : Outport  Port=2
  FC_SUP : Outport  Port=3
  FCE_SUP : Outport  Port=4
  wires:
  Constant10/1 -> Relational Operator4/2
  Constant9/1 -> Relational Operator3/2
  Relational Operator1/1 -> FC_INF/1
  Constant7/1 -> Relational Operator1/2
  Constant8/1 -> Relational Operator2/2
  Relational Operator2/1 -> FCE_INF/1
  Relational Operator3/1 -> FC_SUP/1
  Gain3/1 -> Relational Operator2/1, Relational Operator1/1, Relational Operator3/1, Relational Operator4/1
  tita_hm/1 -> Gain3/1
  Relational Operator4/1 -> FCE_SUP/1

== system planta/Subsystem/Subsystem2 ==
  T_hm* : Inport
  T_tm* : Inport  Port=2
  w_hm : Inport  Port=3
  Subsystem : Subsystem
  Subsystem1 : Subsystem
  T_tm : Outport
  T_hm : Outport  Port=2
  wires:
  Subsystem1/1(T_hm) -> T_hm/1
  T_hm*/1 -> Subsystem1/2(T_hm*)
  w_hm/1 -> Subsystem1/1(w_hm)
  Subsystem/1(T_tm) -> T_tm/1
  T_tm*/1 -> Subsystem/1(T_tm*)

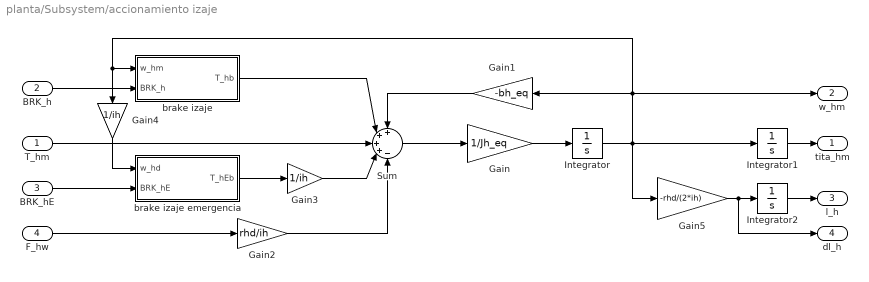
== system planta/Subsystem/accionamiento izaje ==
  T_hm : Inport
  BRK_h : Inport  Port=2
  BRK_hE : Inport  Port=3
  F_hw : Inport  Port=4
  Gain : Gain  Gain=1/Jh_eq
  Gain1 : Gain  Gain=-bh_eq
  Gain2 : Gain  Gain=rhd/ih
  Gain3 : Gain  Gain=1/ih
  Gain4 : Gain  Gain=1/ih
  Gain5 : Gain  Gain=-rhd/(2*ih)
  Integrator : Integrator
  Integrator1 : Integrator  InitialCondition=titahm_0
  Integrator2 : Integrator  InitialCondition=lh_0
  Sum : Sum  Inputs=++++-
  brake izaje : Subsystem
  brake izaje emergencia : Subsystem
  tita_hm : Outport
  w_hm : Outport  Port=2
  l_h : Outport  Port=3
  dl_h : Outport  Port=4
  wires:
  Gain/1 -> Integrator/1
  Sum/1 -> Gain/1
  Gain1/1 -> Sum/1
  F_hw/1 -> Gain2/1
  Integrator/1 -> Gain5/1, brake izaje/1(w_hm), Gain4/1, w_hm/1, Gain1/1, Integrator1/1
  BRK_h/1 -> brake izaje/2(BRK_h)
  BRK_hE/1 -> brake izaje emergencia/2(BRK_hE)
  brake izaje/1(T_hb) -> Sum/2
  T_hm/1 -> Sum/3
  brake izaje emergencia/1(T_hEb) -> Gain3/1
  Gain2/1 -> Sum/5
  Gain3/1 -> Sum/4
  Integrator1/1 -> tita_hm/1
  Gain4/1 -> brake izaje emergencia/1(w_hd)
  Integrator2/1 -> l_h/1
  Gain5/1 -> dl_h/1, Integrator2/1

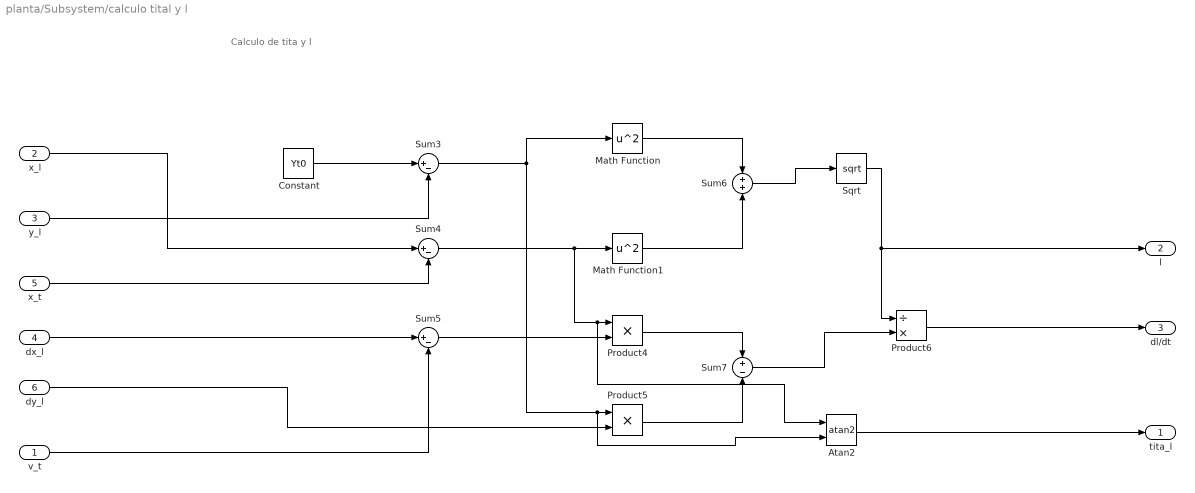
== system planta/Subsystem/calculo tital y l ==
  note: Calculo de tita y l
  v_t : Inport
  x_l : Inport  Port=2
  y_l : Inport  Port=3
  dx_l : Inport  Port=4
  x_t : Inport  Port=5
  dy_l : Inport  Port=6
  Atan2 : Trigonometry  Operator=atan2
  Constant : Constant  Value=Yt0
  Math Function : Math  Operator=square
  Math Function1 : Math  Operator=square
  Product4 : Product
  Product5 : Product
  Product6 : Product  Inputs=/*
  Sqrt : Sqrt
  Sum3 : Sum  Inputs=|+-
  Sum4 : Sum  Inputs=|+-
  Sum5 : Sum  Inputs=|+-
  Sum6 : Sum  Inputs=+|+
  Sum7 : Sum  Inputs=+|-
  tita_l : Outport
  l : Outport  Port=2
  dl/dt : Outport  Port=3
  wires:
  dx_l/1 -> Sum5/1
  y_l/1 -> Sum3/2
  Product4/1 -> Sum7/1
  Constant/1 -> Sum3/1
  Atan2/1 -> tita_l/1
  Sum4/1 -> Atan2/1, Product4/1, Math Function1/1
  x_l/1 -> Sum4/1
  Math Function/1 -> Sum6/1
  Sum7/1 -> Product6/2
  Math Function1/1 -> Sum6/2
  Sum5/1 -> Product4/2
  Sum3/1 -> Atan2/2, Product5/1, Math Function/1
  v_t/1 -> Sum5/2
  Sum6/1 -> Sqrt/1
  dy_l/1 -> Product5/2
  x_t/1 -> Sum4/2
  Product6/1 -> dl/dt/1
  Sqrt/1 -> Product6/1, l/1
  Product5/1 -> Sum7/2

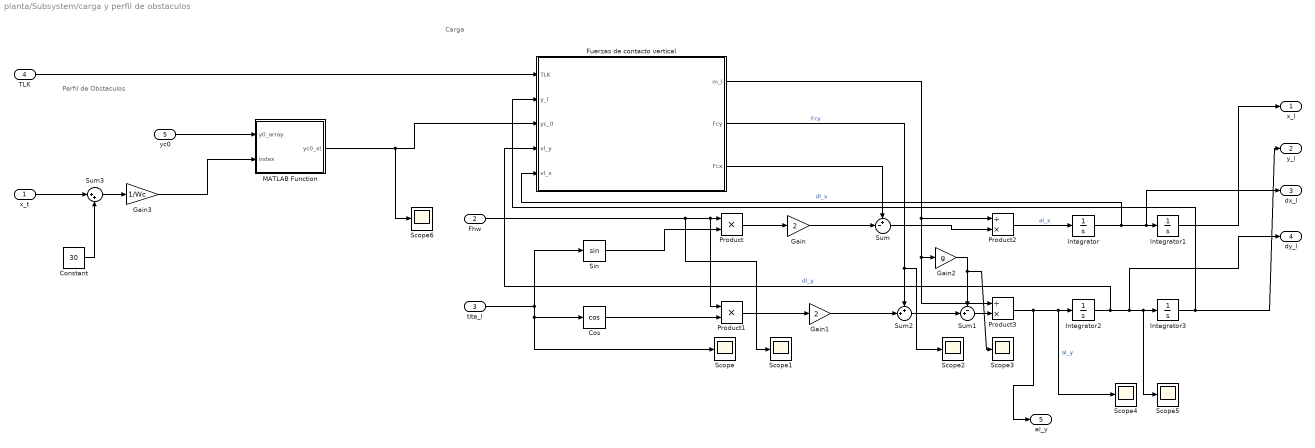
== system planta/Subsystem/carga y perfil de obstaculos ==
  note: Carga
  note: Perfil de Obstaculos
  x_t : Inport
  Fhw : Inport  Port=2
  tita_l : Inport  Port=3
  TLK : Inport  Port=4
  yc0 : Inport  Port=5
  Constant : Constant  Value=30
  Cos : Trigonometry  Operator=cos
  Fuerzas de contacto vertical : Subsystem
  Gain : Gain  Gain=2
  Gain1 : Gain  Gain=2
  Gain2 : Gain  Gain=g
  Gain3 : Gain  Gain=1/Wc
  Integrator : Integrator
  Integrator1 : Integrator  InitialCondition=xl_0
  Integrator2 : Integrator
  Integrator3 : Integrator  InitialCondition=yl_0
  MATLAB Function : MATLAB Function  TreatAsAtomicUnit=on
  Product : Product
  Product1 : Product
  Product2 : Product  Inputs=/*
  Product3 : Product  Inputs=/*
  Scope{,1..6} (7 alike) : Scope
      Scope settings: ActiveDisplayYMinimum=-3.9269908169872414  ActiveDisplayYMaximum=3.9269908169872414  DataLoggingVariableName=ScopeData25
      Scope1 settings: ActiveDisplayYMinimum=-1  ActiveDisplayYMaximum=1  DataLoggingVariableName=ScopeData26
      Scope2 settings: ActiveDisplayYMinimum=12004.689208572614  ActiveDisplayYMaximum=394324.82644801622  DataLoggingVariableName=ScopeData27
      Scope3 settings: DataLoggingVariableName=ScopeData28
      Scope4 settings: ActiveDisplayYMinimum=-65.405205551972983  ActiveDisplayYMaximum=302.48738006597085  DataLoggingVariableName=ScopeData29
      Scope5 settings: ActiveDisplayYMinimum=-0.54307143691279  ActiveDisplayYMaximum=1.0219432569993292  DataLoggingVariableName=ScopeData30
      Scope6 settings: ActiveDisplayYMinimum=-17.482499999999998  ActiveDisplayYMaximum=27.842499999999998  DataLoggingVariableName=ScopeData35
  Sin : Trigonometry
  Sum : Sum  Inputs=+-|
  Sum1 : Sum  Inputs=-+|
  Sum2 : Sum  Inputs=++|
  Sum3 : Sum  Inputs=|++
  x_l : Outport
  y_l : Outport  Port=2
  dx_l : Outport  Port=3
  dy_l : Outport  Port=4
  al_y : Outport  Port=5
  wires:
  tita_l/1 -> Scope/1, Cos/1, Sin/1
  TLK/1 -> Fuerzas de contacto vertical/1(TLK)
  Sum1/1 -> Product3/2
  Constant/1 -> Sum3/2
  Sum/1 -> Product2/2
  Gain/1 -> Sum/2
  Product/1 -> Gain/1
  Integrator3/1 -> Fuerzas de contacto vertical/2(y_l), y_l/1
  Sum2/1 -> Sum1/2
  Gain3/1 -> MATLAB Function/2(index)
  yc0/1 -> MATLAB Function/1(y0_array)
  Integrator2/1 -> Fuerzas de contacto vertical/4(vl_y), dy_l/1, Scope5/1, Integrator3/1  "dl_y"
  Product3/1 -> al_y/1, Scope4/1, Integrator2/1  "al_y"
  Fuerzas de contacto vertical/1(m_l) -> Gain2/1, Product3/1, Product2/1
  Integrator1/1 -> x_l/1
  Fhw/1 -> Scope1/1, Product1/1, Product/1
  Gain1/1 -> Sum2/2
  Product2/1 -> Integrator/1  "al_x"
  MATLAB Function/1(yc0_xt) -> Scope6/1, Fuerzas de contacto vertical/3(yc_0)
  Cos/1 -> Product1/2
  Fuerzas de contacto vertical/3(Fcx) -> Sum/1
  Integrator/1 -> Fuerzas de contacto vertical/5(vl_x), dx_l/1, Integrator1/1  "dl_x"
  Gain2/1 -> Scope3/1, Sum1/1
  x_t/1 -> Sum3/1
  Fuerzas de contacto vertical/2(Fcy) -> Scope2/1, Sum2/1  "Fcy"
  Sum3/1 -> Gain3/1
  Product1/1 -> Gain1/1
  Sin/1 -> Product/2

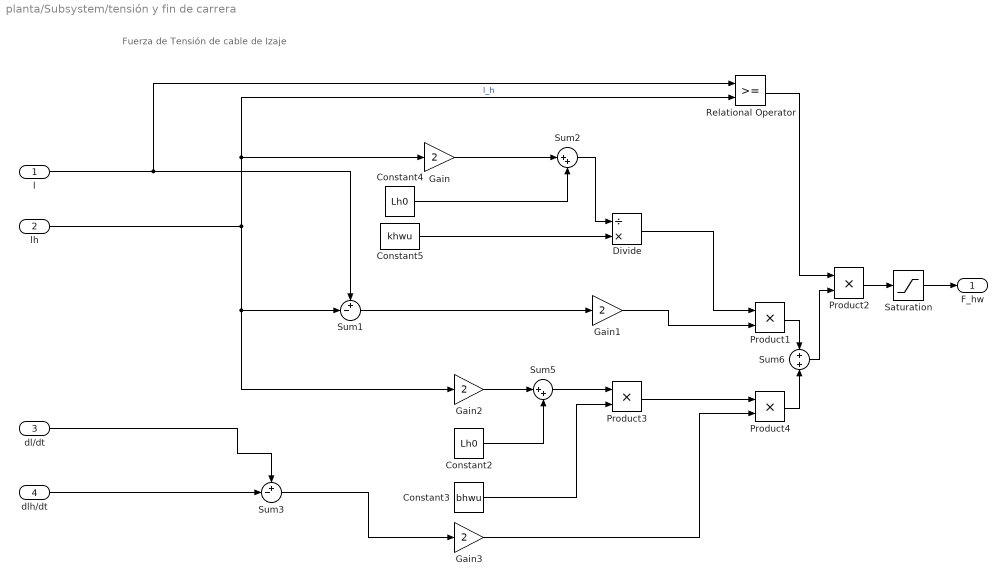
== system planta/Subsystem/tensión y fin de carrera ==
  note: Fuerza de Tensión de cable de Izaje
  l : Inport
  lh : Inport  Port=2
  dl/dt : Inport  Port=3
  dlh/dt : Inport  Port=4
  Constant2 : Constant  Value=Lh0
  Constant3 : Constant  Value=bhwu
  Constant4 : Constant  Value=Lh0
  Constant5 : Constant  Value=khwu
  Divide : Product  Inputs=/*
  Gain{,1..3} (4 alike) : Gain  Gain=2
  Product{1..4} (4 alike) : Product
  Relational Operator : RelationalOperator  OutDataTypeStr=boolean  RndMeth=Simplest  InputSameDT=off
  Saturation : Saturate  UpperLimit=inf  LowerLimit=0
  Sum1 : Sum  Inputs=+-|
  Sum2 : Sum  Inputs=|++
  Sum3 : Sum  Inputs=+-|
  Sum5 : Sum  Inputs=|++
  Sum6 : Sum
  F_hw : Outport
  wires:
  dl/dt/1 -> Sum3/1
  Relational Operator/1 -> Product2/1
  Sum5/1 -> Product3/1
  Sum1/1 -> Gain1/1
  Constant3/1 -> Product3/2
  Product4/1 -> Sum6/2
  Constant4/1 -> Sum2/2
  Product1/1 -> Sum6/1
  dlh/dt/1 -> Sum3/2
  lh/1 -> Relational Operator/2, Gain/1, Gain2/1, Sum1/2  "l_h"
  Product3/1 -> Product4/1
  Constant2/1 -> Sum5/2
  Gain1/1 -> Product1/2
  Gain2/1 -> Sum5/1
  Divide/1 -> Product1/1
  Sum3/1 -> Gain3/1
  Gain3/1 -> Product4/2
  l/1 -> Sum1/1, Relational Operator/1
  Gain/1 -> Sum2/1
  Sum2/1 -> Divide/1
  Constant5/1 -> Divide/2
  Product2/1 -> Saturation/1
  Saturation/1 -> F_hw/1
  Sum6/1 -> Product2/2

== system planta/Subsystem1/Controlador de Velocidad ==
  m_container : Inport
  BRK : Inport  Port=2
  vh_ref : Inport  Port=3
  vh_obs : Inport  Port=4
  Constant : Constant  Value=Ms
  Discrete-Time Integrator : DiscreteIntegrator  IntegratorMethod=Integration: Trapezoidal  ExternalReset=level  SampleTime=-1  ICPrevOutput=DiscIntNeverNeededParam  ICPrevScaledInput=DiscIntNeverNeededParam
  Gain : Gain  Gain=Ki_i
  Gain1 : Gain  Gain=Kp_i
  Gain2 : Gain  Gain=g*rhd/(2*ih)
  Gain3 : Gain  Gain=(2*ih)/rhd
  NOT : Logic  Operator=NOT  IconShape=distinctive  AllPortsSameDT=off  OutDataTypeStr=boolean
  Sum : Sum  Inputs=|++
  Sum1 : Sum  Inputs=+-
  Sum4 : Sum  Inputs=|++
  Sum5 : Sum  Inputs=|++
  T_hm* : Outport
  wires:
  Gain1/1 -> Sum4/1
  Sum1/1 -> Gain3/1
  vh_obs/1 -> Sum1/2
  Gain2/1 -> Sum5/2  "Tg_ff"
  Sum5/1 -> T_hm*/1
  Sum4/1 -> Sum5/1  "T_PID"
  vh_ref/1 -> Sum1/1
  Discrete-Time Integrator/1 -> Gain/1
  Gain/1 -> Sum4/2
  NOT/1 -> Discrete-Time Integrator/2
  BRK/1 -> NOT/1
  Gain3/1 -> Gain1/1, Discrete-Time Integrator/1  "e_wh"
  Sum/1 -> Gain2/1
  m_container/1 -> Sum/1
  Constant/1 -> Sum/2

== system planta/Subsystem1/Modulación de la Referencia ==
  vh : Inport
  Rate Limiter : RateLimiter  RisingSlewLimit=ah_max  FallingSlewLimit=-ah_max  SampleTimeMode=inherited  InitialCondition=vh_0
  Saturation : Saturate  UpperLimit=vh_max  LowerLimit=-vh_max
  vh_ref : Outport
  wires:
  Rate Limiter/1 -> vh_ref/1
  vh/1 -> Saturation/1
  Saturation/1 -> Rate Limiter/1

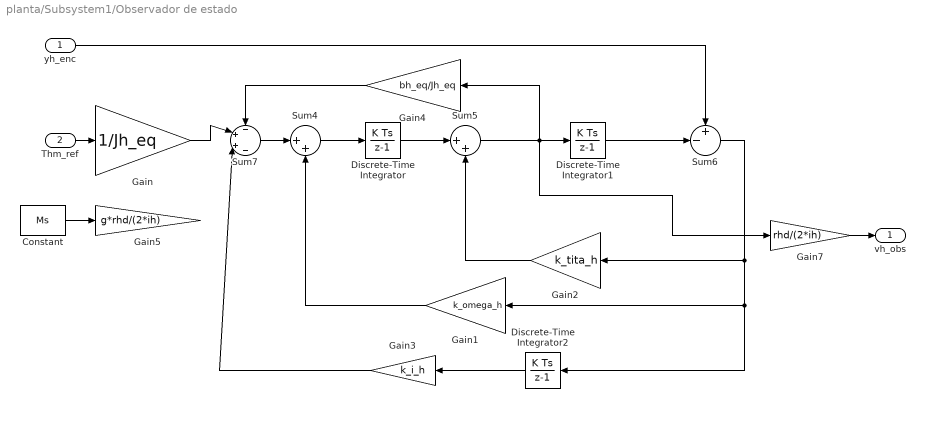
== system planta/Subsystem1/Observador de estado ==
  yh_enc : Inport
  Thm_ref : Inport  Port=2
  Constant : Constant  Value=Ms
  Discrete-Time Integrator : DiscreteIntegrator  SampleTime=-1  ICPrevOutput=DiscIntNeverNeededParam  ICPrevScaledInput=DiscIntNeverNeededParam
  Discrete-Time Integrator1 : DiscreteIntegrator  InitialCondition=titahm_0  SampleTime=-1  ICPrevOutput=DiscIntNeverNeededParam  ICPrevScaledInput=DiscIntNeverNeededParam
  Discrete-Time Integrator2 : DiscreteIntegrator  SampleTime=-1  ICPrevOutput=DiscIntNeverNeededParam  ICPrevScaledInput=DiscIntNeverNeededParam
  Gain : Gain  Gain=1/Jh_eq
  Gain1 : Gain  Gain=k_omega_h
  Gain2 : Gain  Gain=k_tita_h
  Gain3 : Gain  Gain=k_i_h
  Gain4 : Gain  Gain=bh_eq/Jh_eq
  Gain5 : Gain  Gain=g*rhd/(2*ih)
  Gain7 : Gain  Gain=rhd/(2*ih)
  Sum4 : Sum  Inputs=|++
  Sum5 : Sum  Inputs=|++
  Sum6 : Sum  Inputs=+-|
  Sum7 : Sum  Inputs=-++-
  vh_obs : Outport
  wires:
  Thm_ref/1 -> Gain/1
  Gain1/1 -> Sum4/2
  Sum7/1 -> Sum4/1
  Sum5/1 -> Gain4/1, Gain7/1, Discrete-Time Integrator1/1
  Discrete-Time Integrator1/1 -> Sum6/2
  Sum6/1 -> Discrete-Time Integrator2/1, Gain1/1, Gain2/1
  Discrete-Time Integrator2/1 -> Gain3/1
  Gain2/1 -> Sum5/2
  Discrete-Time Integrator/1 -> Sum5/1
  Sum4/1 -> Discrete-Time Integrator/1
  Gain3/1 -> Sum7/3
  Gain/1 -> Sum7/2
  Gain4/1 -> Sum7/1
  Constant/1 -> Gain5/1
  yh_enc/1 -> Sum6/1
  Gain7/1 -> vh_obs/1

== system planta/Subsystem2/Control de Balanceo ==
  anti-sway : Inport
  yh_enc : Inport  Port=2
  tita_l : Inport  Port=3
  Abs : Abs  SaturateOnIntegerOverflow=off
  Constant : Constant  Value=Yt0
  Gain : Gain  Gain=g
  Gain1 : Gain  Gain=2
  Product : Product  Inputs=3
  Sqrt : Sqrt
  Sum : Sum  Inputs=|+-
  ζ : Gain  Gain=zitta
  v_sway : Outport
  wires:
  Sqrt/1 -> ζ/1
  Product/1 -> v_sway/1
  Abs/1 -> Sqrt/1
  Gain/1 -> Abs/1
  tita_l/1 -> Product/1
  ζ/1 -> Gain1/1
  anti-sway/1 -> Product/3
  Gain1/1 -> Product/2
  Sum/1 -> Gain/1
  Constant/1 -> Sum/1
  yh_enc/1 -> Sum/2

== system planta/Subsystem2/Controlador de Velocidad ==
  BRK_t : Inport
  vt_ref : Inport  Port=2
  vt_obs : Inport  Port=3
  Discrete-Time Integrator : DiscreteIntegrator  IntegratorMethod=Integration: Trapezoidal  ExternalReset=level  SampleTime=-1  ICPrevOutput=DiscIntNeverNeededParam  ICPrevScaledInput=DiscIntNeverNeededParam
  Gain5 : Gain  Gain=Ki_c
  Gain6 : Gain  Gain=Kp_c
  NOT : Logic  Operator=NOT  IconShape=distinctive  AllPortsSameDT=off  OutDataTypeStr=boolean
  Sum6 : Sum  Inputs=+-
  Sum7 : Sum  Inputs=++|
  T_tm* : Outport
  wires:
  Sum6/1 -> Gain6/1, Discrete-Time Integrator/1  "e_v"
  Sum7/1 -> T_tm*/1
  Gain5/1 -> Sum7/2
  vt_ref/1 -> Sum6/1
  Gain6/1 -> Sum7/1
  vt_obs/1 -> Sum6/2
  Discrete-Time Integrator/1 -> Gain5/1
  BRK_t/1 -> NOT/1
  NOT/1 -> Discrete-Time Integrator/2

== system planta/Subsystem2/Corrección de Referencia ==
  vx_cmd : Inport
  v_sway : Inport  Port=2
  Rate Limiter : RateLimiter  RisingSlewLimit=at_max  FallingSlewLimit=-at_max  SampleTimeMode=inherited  InitialCondition=vt_0
  Saturation : Saturate  UpperLimit=vt_max  LowerLimit=-vt_max
  Sum1 : Sum  Inputs=++|
  vt_ref : Outport
  wires:
  v_sway/1 -> Sum1/2
  Saturation/1 -> Rate Limiter/1
  Rate Limiter/1 -> vt_ref/1
  Sum1/1 -> Saturation/1  "vt_cmd"
  vx_cmd/1 -> Sum1/1

== system planta/Subsystem2/Observador de estado ==
  Ttm_ref : Inport
  tita_tm_enc : Inport  Port=2
  Delay One Step1 : Delay  Commented=through  DelayLength=1  InitialCondition=xtd_0
  Discrete-Time Integrator : DiscreteIntegrator  SampleTime=-1  ICPrevOutput=DiscIntNeverNeededParam  ICPrevScaledInput=DiscIntNeverNeededParam
  Discrete-Time Integrator1 : DiscreteIntegrator  InitialCondition=titatm_0  SampleTime=-1  ICPrevOutput=DiscIntNeverNeededParam  ICPrevScaledInput=DiscIntNeverNeededParam
  Discrete-Time Integrator2 : DiscreteIntegrator  SampleTime=-1  ICPrevOutput=DiscIntNeverNeededParam  ICPrevScaledInput=DiscIntNeverNeededParam
  Gain : Gain  Gain=1/Jt_eq
  Gain1 : Gain  Gain=k_omega_c
  Gain2 : Gain  Gain=k_tita_c
  Gain3 : Gain  Gain=k_i_c
  Gain4 : Gain  Gain=rtd/it
  Sum4 : Sum  Inputs=|++
  Sum5 : Sum  Inputs=|++
  Sum6 : Sum  Inputs=+-|
  Sum7 : Sum  Inputs=|++
  vt_obs : Outport
  wires:
  Discrete-Time Integrator/1 -> Sum5/1
  Sum4/1 -> Discrete-Time Integrator/1
  tita_tm_enc/1 -> Delay One Step1/1
  Discrete-Time Integrator2/1 -> Gain3/1
  Gain1/1 -> Sum4/2
  Sum6/1 -> Discrete-Time Integrator2/1, Gain1/1, Gain2/1
  Discrete-Time Integrator1/1 -> Sum6/2
  Sum7/1 -> Sum4/1
  Gain3/1 -> Sum7/2
  Gain/1 -> Sum7/1
  Gain2/1 -> Sum5/2
  Ttm_ref/1 -> Gain/1
  Sum5/1 -> Gain4/1, Discrete-Time Integrator1/1
  Delay One Step1/1 -> Sum6/1
  Gain4/1 -> vt_obs/1

== system planta/Subsystem/Carro/Subsystem ==
  BRK_t : Inport
  w_tm : Inport  Port=2
  Constant : Constant  Value=0
  Gain1 : Gain  Gain=-Ttb_Max
  Gain8 : Gain  Gain=btb
  Switch : Switch  Criteria=u2 ~= 0  SaturateOnIntegerOverflow=off  InputSameDT=off
  Tanh : Trigonometry  Operator=tanh
  T_tb : Outport
  wires:
  Constant/1 -> Switch/1
  BRK_t/1 -> Switch/2
  Switch/1 -> T_tb/1  "T_tb"
  w_tm/1 -> Gain8/1
  Gain8/1 -> Tanh/1
  Tanh/1 -> Gain1/1
  Gain1/1 -> Switch/3

== system planta/Subsystem/Subsystem2/Subsystem ==
  T_tm* : Inport
  Constant : Constant  Value=Ttm_Max
  Constant1 : Constant  Value=-Ttm_Max
  Gain : Gain  Gain=1/tau_tm
  Integrator : Integrator
  Max : MinMax  Function=max  Inputs=2
  Min : MinMax  Inputs=2
  Sum : Sum  Inputs=|+-
  Zero-Order Hold : ZeroOrderHold  SampleTime=tau_tm
  T_tm : Outport
  wires:
  Min/1 -> Sum/1
  Gain/1 -> Integrator/1
  Sum/1 -> Gain/1
  Integrator/1 -> Sum/2, T_tm/1
  Max/1 -> Min/2
  Constant/1 -> Min/1
  Constant1/1 -> Max/1
  T_tm*/1 -> Zero-Order Hold/1
  Zero-Order Hold/1 -> Max/2

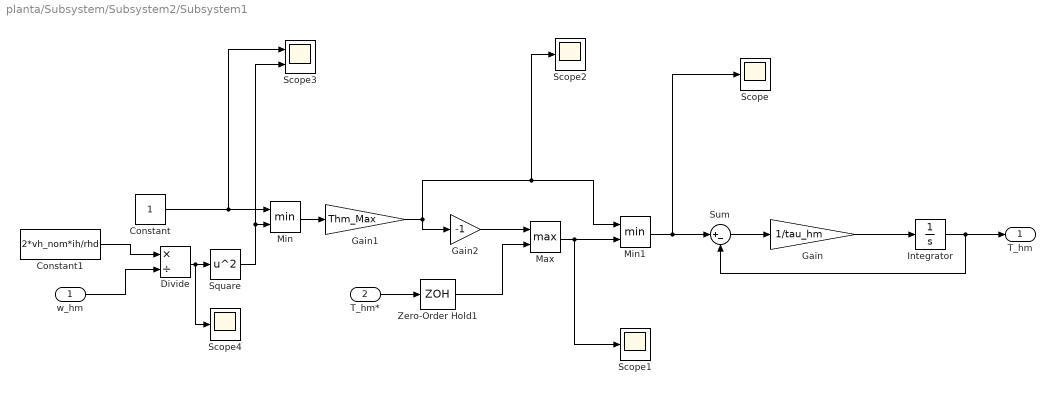
== system planta/Subsystem/Subsystem2/Subsystem1 ==
  w_hm : Inport
  T_hm* : Inport  Port=2
  Constant : Constant
  Constant1 : Constant  Value=2*vh_nom*ih/rhd
  Divide : Product  Inputs=*/
  Gain : Gain  Gain=1/tau_hm
  Gain1 : Gain  Gain=Thm_Max
  Gain2 : Gain  Gain=-1
  Integrator : Integrator
  Max : MinMax  Function=max  Inputs=2
  Min : MinMax  Inputs=2
  Min1 : MinMax  Inputs=2
  Scope{,1..2,4} (4 alike) : Scope
      Scope settings: ActiveDisplayYMinimum=-2500  ActiveDisplayYMaximum=22500  DataLoggingVariableName=ScopeData3
      Scope1 settings: ActiveDisplayYMinimum=-2500  ActiveDisplayYMaximum=22500  DataLoggingVariableName=ScopeData4
      Scope2 settings: ActiveDisplayYMinimum=481.45655  ActiveDisplayYMaximum=22168.72705  DataLoggingVariableName=ScopeData5
      Scope4 settings: ActiveDisplayYMinimum=-0.06596  ActiveDisplayYMaximum=-0.00953  DataLoggingVariableName=ScopeData7
  Scope3 : Scope  NumInputPorts=2
      settings: ActiveDisplayYMinimum=-9.1717430786370772E+28  ActiveDisplayYMaximum=8.25456877077337E+29  DataLoggingVariableName=ScopeData6
  Square : Math  Operator=square
  Sum : Sum  Inputs=|+-
  Zero-Order Hold1 : ZeroOrderHold  SampleTime=tau_hm
  T_hm : Outport
  wires:
  Sum/1 -> Gain/1
  Gain/1 -> Integrator/1
  Integrator/1 -> Sum/2, T_hm/1
  Constant/1 -> Scope3/1, Min/1
  w_hm/1 -> Divide/2
  Constant1/1 -> Divide/1
  Divide/1 -> Scope4/1, Square/1
  Square/1 -> Scope3/2, Min/2
  Min/1 -> Gain1/1
  Gain1/1 -> Scope2/1, Min1/1, Gain2/1
  T_hm*/1 -> Zero-Order Hold1/1
  Gain2/1 -> Max/1
  Max/1 -> Scope1/1, Min1/2
  Min1/1 -> Scope/1, Sum/1
  Zero-Order Hold1/1 -> Max/2

== system planta/Subsystem/accionamiento izaje/brake izaje ==
  w_hm : Inport
  BRK_h : Inport  Port=2
  Constant : Constant  Value=0
  Gain : Gain  Gain=bhb
  Gain1 : Gain  Gain=-Thb_Max
  Switch : Switch  Criteria=u2 ~= 0  SaturateOnIntegerOverflow=off  InputSameDT=off
  Tanh : Trigonometry  Operator=tanh
  T_hb : Outport
  wires:
  Switch/1 -> T_hb/1
  Constant/1 -> Switch/1
  BRK_h/1 -> Switch/2
  w_hm/1 -> Gain/1
  Gain/1 -> Tanh/1
  Tanh/1 -> Gain1/1
  Gain1/1 -> Switch/3

== system planta/Subsystem/accionamiento izaje/brake izaje emergencia ==
  w_hd : Inport
  BRK_hE : Inport  Port=2
  Constant : Constant  Value=0
  Gain : Gain  Gain=bhEb
  Gain1 : Gain  Gain=-ThEb_Max
  Switch : Switch  Criteria=u2 ~= 0  SaturateOnIntegerOverflow=off  InputSameDT=off
  Tanh : Trigonometry  Operator=tanh
  T_hEb : Outport
  wires:
  Tanh/1 -> Gain1/1
  Gain/1 -> Tanh/1
  Constant/1 -> Switch/1
  w_hd/1 -> Gain/1
  Switch/1 -> T_hEb/1
  BRK_hE/1 -> Switch/2
  Gain1/1 -> Switch/3

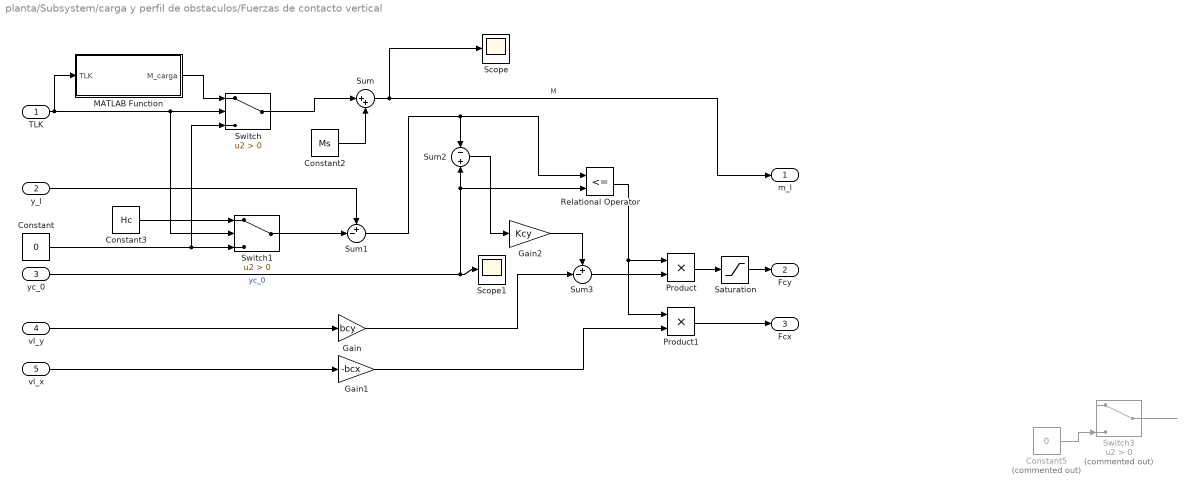
== system planta/Subsystem/carga y perfil de obstaculos/Fuerzas de contacto vertical ==
  TLK : Inport
  y_l : Inport  Port=2
  yc_0 : Inport  Port=3
  vl_y : Inport  Port=4
  vl_x : Inport  Port=5
  Constant : Constant  Value=0
  Constant2 : Constant  Value=Ms
  Constant3 : Constant  Value=Hc
  Constant5 : Constant  Commented=on  Value=0
  Gain : Gain  Gain=bcy
  Gain1 : Gain  Gain=-bcx
  Gain2 : Gain  Gain=Kcy
  MATLAB Function : MATLAB Function  TreatAsAtomicUnit=on
  Product : Product
  Product1 : Product
  Relational Operator : RelationalOperator  Operator=<=  OutDataTypeStr=boolean  RndMeth=Simplest  InputSameDT=off
  Saturation : Saturate  UpperLimit=inf  LowerLimit=0
  Scope : Scope
      settings: ActiveDisplayYMinimum=-30040.049311756404  ActiveDisplayYMaximum=65258.780060315854  DataLoggingVariableName=ScopeData31
  Scope1 : Scope
      settings: ActiveDisplayYMinimum=12.776564460216019  ActiveDisplayYMaximum=15.5369149188378  DataLoggingVariableName=ScopeData32
  Sum : Sum  Inputs=|++
  Sum1 : Sum  Inputs=+-|
  Sum2 : Sum  Inputs=-|+
  Sum3 : Sum  Inputs=+-|
  Switch : Switch  Criteria=u2 > Threshold  SaturateOnIntegerOverflow=off  InputSameDT=off
  Switch1 : Switch  Criteria=u2 > Threshold  SaturateOnIntegerOverflow=off  InputSameDT=off
  Switch3 : Switch  Commented=on  Criteria=u2 > Threshold  SaturateOnIntegerOverflow=off  InputSameDT=off
  m_l : Outport
  Fcy : Outport  Port=2
  Fcx : Outport  Port=3
  wires:
  TLK/1 -> MATLAB Function/1(TLK), Switch1/2, Switch/2
  Constant/1 -> Switch1/3, Switch/3
  Constant3/1 -> Switch1/1
  Switch/1 -> Sum/1
  Sum/1 -> Scope/1, m_l/1  "M"
  Constant2/1 -> Sum/2
  Switch1/1 -> Sum1/2
  y_l/1 -> Sum1/1
  Sum1/1 -> Relational Operator/1, Sum2/1
  yc_0/1 -> Scope1/1, Sum2/2, Relational Operator/2  "yc_0"
  Sum2/1 -> Gain2/1
  Gain2/1 -> Sum3/1
  Relational Operator/1 -> Product1/1, Product/1
  Product1/1 -> Fcx/1
  Gain/1 -> Sum3/2
  vl_y/1 -> Gain/1
  vl_x/1 -> Gain1/1
  Gain1/1 -> Product1/2
  Sum3/1 -> Product/2
  Constant5/1 -> Switch3/3
  Switch3/1 -> ?
  ? -> Switch3/1, Switch3/2
  Product/1 -> Saturation/1
  Saturation/1 -> Fcy/1
  MATLAB Function/1(M_carga) -> Switch/1

== matlab function planta/Subsystem/carga y perfil de obstaculos/MATLAB Function ==
  data: y0_array input; yc0_xt output; index input
function yc0_xt= calcula_y0(y0_array,index)
index = floor(index)+1;
index = min(max(index,1),33);
yc0_xt = y0_array(index);
